simulink model "MLDDPG_GL_vhold_raskovav2"  (R2025b)
settings: Solver=ode4  StartTime=0.0  StopTime=tml  FixedStep=dtml  RelTol=1e-3
undefined symbols (not defined in the file or in its folder): denlong, DiscIntNeverNeededParam, numlong
libraries: simulink x3, rllib x1, simulink_extras x1
settings Model: Creator=gflla  LastModifiedBy=gflla

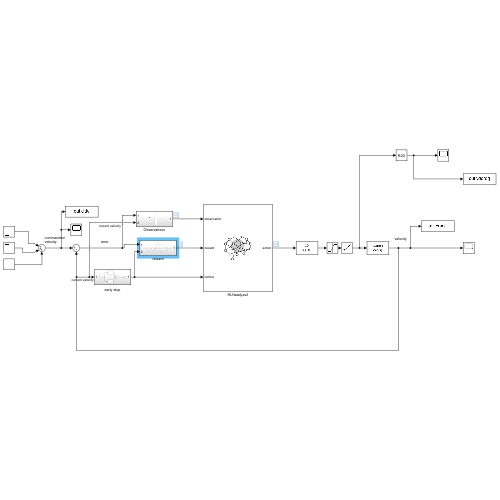
[thumbnail: Simulink's stored preview of the top-level diagram]
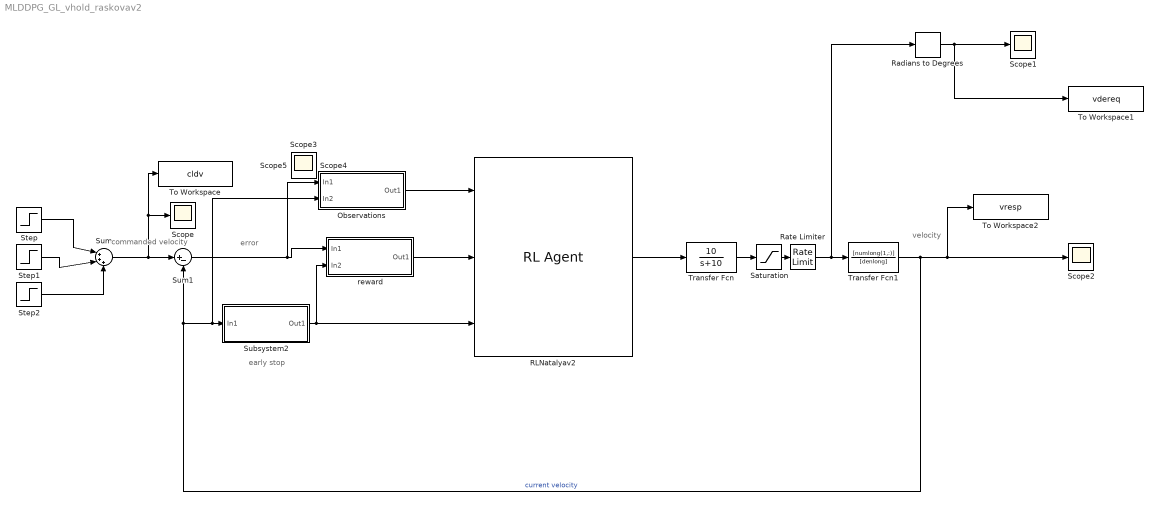
== system MLDDPG_GL_vhold_raskovav2 ==
  note: early stop
  note: error
  note: commanded
      | velocity
  note: velocity
  Observations : Subsystem
  RLNatalyav2 : rllib/RL Agent  Agent=agentNatalyav2  ExternalActionAsInput=off  ProvideLastAction=off  ProvideCumRwd=off  TreatAsDirectFeedthrough=on  UseStrictObservationDataTypes=off
  Radians to Degrees : simulink_extras/Transformations/Radians to Degrees
  Rate Limiter : RateLimiter  RisingSlewLimit=20*pi/180  FallingSlewLimit=-20*pi/180  SampleTimeMode=inherited
  Saturation : Saturate  UpperLimit=20*pi/180  LowerLimit=-20*pi/180
  Scope{,1..5} (6 alike) : Scope
      Scope settings: ActiveDisplayYMinimum=-2.3187439905239677  ActiveDisplayYMaximum=2.4944944768582045
      Scope1 settings: ActiveDisplayYMinimum=-25.944192470061541  ActiveDisplayYMaximum=25.873926983917425
      Scope2 settings: ActiveDisplayYMinimum=-8.9794745537609746  ActiveDisplayYMaximum=11.230818477730748  DataLoggingVariableName=ScopeData2
      Scope3 settings: ActiveDisplayYMinimum=3.6203416674662741  ActiveDisplayYMaximum=68.122340541740371  DataLoggingVariableName=ScopeData3
      Scope4 settings: ActiveDisplayYMinimum=-7.59967109131441  ActiveDisplayYMaximum=5.2925072330415412  DataLoggingVariableName=ScopeData4
      Scope5 settings: DataLoggingVariableName=ScopeData5
  Step : Step  After=2  SampleTime=0
  Step1 : Step  Time=2  Before=2  After=-2  SampleTime=0
  Step2 : Step  Time=3  Before=-2  After=0  SampleTime=0
  Subsystem2 : Subsystem
  Sum : Sum  Inputs=|+++
  Sum1 : Sum  Inputs=|+-
  To Workspace : ToWorkspace  VariableName=cldv  SaveFormat=Timeseries  SampleTime=-1
  To Workspace1 : ToWorkspace  VariableName=vdereq  SaveFormat=Timeseries  SampleTime=-1
  To Workspace2 : ToWorkspace  VariableName=vresp  SaveFormat=Timeseries  SampleTime=-1
  Transfer Fcn : TransferFcn  Numerator=[10]  Denominator=[1 10]
  Transfer Fcn1 : TransferFcn  Numerator=[numlong(1,:)]  Denominator=[denlong]
  reward : Subsystem
  wires:
  Step/1 -> Sum/1
  Step1/1 -> Sum/2
  Step2/1 -> Sum/3
  Transfer Fcn/1 -> Saturation/1
  Sum/1 -> Sum1/1, To Workspace/1, Scope/1
  Saturation/1 -> Rate Limiter/1
  Rate Limiter/1 -> Radians to Degrees/1, Transfer Fcn1/1
  Transfer Fcn1/1 -> Observations/2(In2), Subsystem2/1(In1), Sum1/2, To Workspace2/1, Scope2/1  "current velocity"
  Radians to Degrees/1 -> To Workspace1/1, Scope1/1
  RLNatalyav2/1 -> Transfer Fcn/1
  Sum1/1 -> reward/1(In1), Observations/1(In1)
  Subsystem2/1(Out1) -> RLNatalyav2/3, reward/2(In2)
  Observations/1(Out1) -> RLNatalyav2/1
  reward/1(Out1) -> RLNatalyav2/2

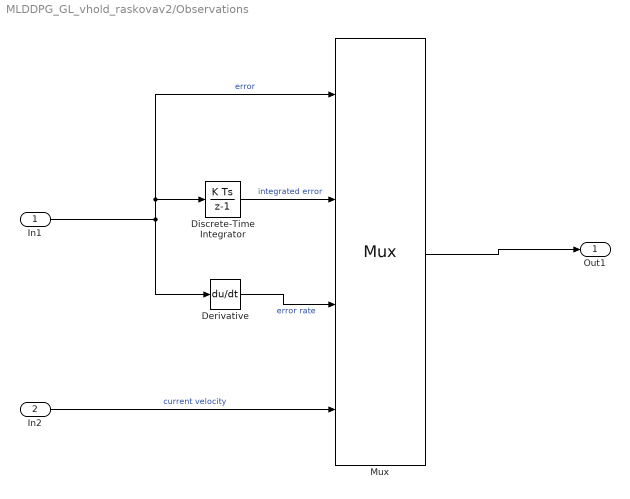
== system MLDDPG_GL_vhold_raskovav2/Observations ==
  In1 : Inport
  In2 : Inport  Port=2
  Derivative : Derivative
  Discrete-Time Integrator : DiscreteIntegrator  SampleTime=-1  ICPrevOutput=DiscIntNeverNeededParam  ICPrevScaledInput=DiscIntNeverNeededParam
  Mux : Mux
  Out1 : Outport
  wires:
  In1/1 -> Derivative/1, Discrete-Time Integrator/1, Mux/1  "error"
  Derivative/1 -> Mux/3  "error rate"
  Discrete-Time Integrator/1 -> Mux/2  "integrated error"
  Mux/1 -> Out1/1
  In2/1 -> Mux/4  "current velocity"

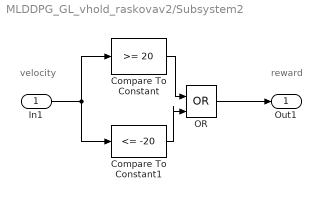
== system MLDDPG_GL_vhold_raskovav2/Subsystem2 ==
  note: reward
  note: velocity
  In1 : Inport
  Compare To Constant : simulink/Logic and Bit Operations/Compare To Constant  relop=>=  const=20  OutDataTypeStr=boolean
  Compare To Constant1 : simulink/Logic and Bit Operations/Compare To Constant  relop=<=  const=-20  OutDataTypeStr=boolean
  OR : Logic  Operator=OR  IconShape=distinctive  AllPortsSameDT=off  OutDataTypeStr=boolean
  Out1 : Outport
  wires:
  In1/1 -> Compare To Constant1/1, Compare To Constant/1
  Compare To Constant/1 -> OR/1
  Compare To Constant1/1 -> OR/2
  OR/1 -> Out1/1

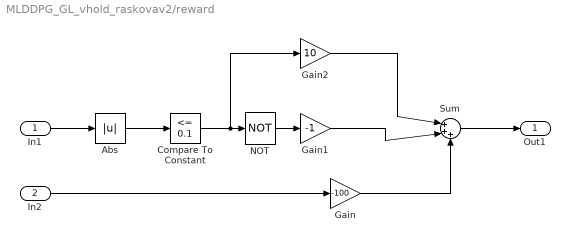
== system MLDDPG_GL_vhold_raskovav2/reward ==
  In1 : Inport
  In2 : Inport  Port=2
  Abs : Abs  SaturateOnIntegerOverflow=off
  Compare To Constant : simulink/Logic and Bit Operations/Compare To Constant  relop=<=  const=0.1  OutDataTypeStr=boolean
  Gain : Gain  Gain=-100
  Gain1 : Gain  Gain=-1
  Gain2 : Gain  Gain=10
  NOT : Logic  Operator=NOT  IconShape=distinctive  AllPortsSameDT=off  OutDataTypeStr=boolean
  Sum : Sum  Inputs=|+++
  Out1 : Outport
  wires:
  In2/1 -> Gain/1
  Sum/1 -> Out1/1
  In1/1 -> Abs/1
  Abs/1 -> Compare To Constant/1
  Compare To Constant/1 -> Gain2/1, NOT/1
  NOT/1 -> Gain1/1
  Gain2/1 -> Sum/1
  Gain/1 -> Sum/3
  Gain1/1 -> Sum/2
